simulink model "FsaeDynoFull"  (R2026a)
settings: Solver=FixedStepDiscrete  StopTime=t_stop  FixedStep=Ts  EnableMultiTasking=on
PreLoadFcn:
  | FsaeDynoFullData;
InitFcn:
  | FsaeDynoFullData;
values from neighbouring files (symbols this model uses):
  ce = 100    [FsaeDynoFullData.m]
  k_pre = 0.95    [FsaeDynoFullData.m]    (also in FsaeDynoFullPlot.m = evalin('base','k_pre'))
  Ki_id = Rs*wc_dut    (= 13.3454855924)    [FsaeDynoFullData.m]
  Ki_ids = Rs_y*wc_load    (= 47.1238898038)    [FsaeDynoFullData.m]
  Ki_iq = Rs*wc_dut    (= 13.3454855924)    [FsaeDynoFullData.m]
  Ki_iqs = Rs_y*wc_load    (= 47.1238898038)    [FsaeDynoFullData.m]
  Kp_id = Ld*wc_dut    (= 0.102541584213)    [FsaeDynoFullData.m]
  Kp_ids = Ld_y*wc_load    (= 0.204203522483)    [FsaeDynoFullData.m]
  Kp_iq = Lq*wc_dut    (= 0.105557513161)    [FsaeDynoFullData.m]
  Kp_iqs = Lq_y*wc_load    (= 0.204203522483)    [FsaeDynoFullData.m]
  Ld = 40.8e-6    (= 4.08e-05)    [FsaeDynoFullData.m]
  Lq = 42.0e-6    (= 4.2e-05)    [FsaeDynoFullData.m]
  p = 10    [FsaeDynoFullData.m]    (also in buildFsaeDynoFull.m = get_param(ss,'PortHandles'))
  psim = 0.03095    [FsaeDynoFullData.m]
  R_dis_dut = 1/G_dis_dut  - R_disRly    [FsaeDynoFullData.m]
  R_dis_load = 1/G_dis_load - R_disRly    [FsaeDynoFullData.m]
  R_pre_dut = fzero(@(R) preErr(R, Cdc_dut,  G_leak_dut  + G_disRlyOff), [1 1e5])    [FsaeDynoFullData.m]
  R_pre_load = fzero(@(R) preErr(R, Cdc_load, G_leak_load + G_disRlyOff), [1 1e5])    [FsaeDynoFullData.m]
  R_stby_dut = 50e3    (= 50000)    [FsaeDynoFullData.m]
  R_stby_load = 50e3    (= 50000)    [FsaeDynoFullData.m]
  t_InvEnDelay = 0.05    [FsaeDynoFullData.m]
  t_TSoff = t_test + 0.8 + 0.7    (= 2.7)    [FsaeDynoFullData.m]    (also in FsaeDynoFullPlot.m = evalin('base','t_TSoff'))
  Ts = 1e-5    (= 1e-05)    [FsaeDynoFullData.m]
  VbattMin = 50    [FsaeDynoFullData.m]
  VDC_VECT = Vnom*[0.9 1.0 1.1]    [FsaeDynoFullData.m]
  Vnom2 = 400    [FsaeDynoFullData.m]
libraries: nesl_utility x37, fl_lib x22, ee_lib x22, simulink x4, eeTransforms x2, batteryecm_lib x2, eePmsmFieldOrientedControl x1, eePmsmCurrentController x1, eePmsmCurrentReferenceGen x1, eePmsmTorqueEstimator x1, eePwmGeneratorTwoLevel x1
(part 2 of 2)

== system FsaeDynoFull/Sensing Torque IPMSM ==
  Elastic Coupling : fl_lib/Mechanical/Rotational Elements/Rotational Damper  D=ce N*m/(rad/s)  w_specify=off  w_priority=None  w=0 rad/s  w_nominal_specify=off  w_nominal_value=1  w_nominal_unit=rad/s  t_specify=off  t_priority=None  t=0 N*m  t_nominal_specify=off  t_nominal_value=1  t_nominal_unit=N*m
      settings: LogSimulationData=on
  Goto3 : Goto  TagVisibility=global
  Mechanical Rotational Reference1 : fl_lib/Mechanical/Rotational Elements/Mechanical Rotational Reference
  PS-Simulink Converter1 : nesl_utility/PS-Simulink Converter  PhysicalDomain=network_engine_domain  SubClassName=ps_output  LeftPortType=input  RightPortType=output  PseudoPeriodic=off  Frequencies=[]  VectorFormat=1-D array  Unit=rad/s  AffineConversion=off
  PS-Simulink Converter2 : nesl_utility/PS-Simulink Converter  PhysicalDomain=network_engine_domain  SubClassName=ps_output  LeftPortType=input  RightPortType=output  PseudoPeriodic=off  Frequencies=[]  VectorFormat=1-D array  Unit=rad  AffineConversion=off
  PS-Simulink Converter3 : nesl_utility/PS-Simulink Converter  PhysicalDomain=network_engine_domain  SubClassName=ps_output  LeftPortType=input  RightPortType=output  PseudoPeriodic=off  Frequencies=[]  VectorFormat=1-D array  Unit=N*m  AffineConversion=off
  Rotational Motion Sensor : fl_lib/Mechanical/Mechanical Sensors/Ideal Rotational Motion Sensor  reference=foundation.enum.MeasurementReference.difference  acceleration_port=false  velocity_port=true  position_port=true  wrap_angle=simscape.enum.onoff.off  offset=0 deg
  Torque Sensor : fl_lib/Mechanical/Mechanical Sensors/Ideal Torque Sensor
  R : PMIOPort  Side=Left
  C : PMIOPort  Port=2  Side=Right
  tag scope: Tq_meas=global, W=global
  wires:
  PS-Simulink Converter2/1 -> Goto3/1
  PS-Simulink Converter1/1 -> [W]
  PS-Simulink Converter3/1 -> [Tq_meas]
  connections:
  Mechanical Rotational Reference1/LConn1 -- Rotational Motion Sensor/RConn1
  Rotational Motion Sensor/RConn3 -- PS-Simulink Converter2/LConn1
  Rotational Motion Sensor/RConn2 -- PS-Simulink Converter1/LConn1
  Torque Sensor/RConn2 -- PS-Simulink Converter3/LConn1
  Torque Sensor/RConn1 -- Elastic Coupling/LConn1 -- Rotational Motion Sensor/LConn1
  Elastic Coupling/RConn1 -- C/RConn1
  Torque Sensor/LConn1 -- R/RConn1

== system FsaeDynoFull/Sensing Torque IPMSM1 ==
  PS-Simulink Converter3 : nesl_utility/PS-Simulink Converter  PhysicalDomain=network_engine_domain  SubClassName=ps_output  LeftPortType=input  RightPortType=output  PseudoPeriodic=off  Frequencies=[]  VectorFormat=1-D array  Unit=N*m  AffineConversion=off
  Torque Sensor : fl_lib/Mechanical/Mechanical Sensors/Ideal Torque Sensor
  C : PMIOPort  Side=Left
  R : PMIOPort  Port=2  Side=Right
  tag scope: Tq_asm=global
  wires:
  PS-Simulink Converter3/1 -> [Tq_asm]
  connections:
  C/RConn1 -- Torque Sensor/RConn1
  R/RConn1 -- Torque Sensor/LConn1
  Torque Sensor/RConn2 -- PS-Simulink Converter3/LConn1

== system FsaeDynoFull/Sensing current1 ==
  Current Sensor : ee_lib/Sensors & Transducers/Current Sensor (Three-Phase)  port_option=ee.enum.threePhasePort.composite
  PS-Simulink Converter : nesl_utility/PS-Simulink Converter  PhysicalDomain=network_engine_domain  SubClassName=ps_output  LeftPortType=input  RightPortType=output  PseudoPeriodic=off  Frequencies=[]  VectorFormat=1-D array  Unit=A  AffineConversion=off
  1 : PMIOPort  Side=Left
  2 : PMIOPort  Port=2  Side=Right
  tag scope: I_ABC=global
  wires:
  PS-Simulink Converter/1 -> [I_ABC]
  connections:
  1/RConn1 -- Current Sensor/LConn1
  2/RConn1 -- Current Sensor/RConn2
  Current Sensor/RConn1 -- PS-Simulink Converter/LConn1

== system FsaeDynoFull/Sensing current2 ==
  Current Sensor : ee_lib/Sensors & Transducers/Current Sensor (Three-Phase)  port_option=ee.enum.threePhasePort.composite
  PS-Simulink Converter : nesl_utility/PS-Simulink Converter  PhysicalDomain=network_engine_domain  SubClassName=ps_output  LeftPortType=input  RightPortType=output  PseudoPeriodic=off  Frequencies=[]  VectorFormat=1-D array  Unit=A  AffineConversion=off
  1 : PMIOPort  Side=Left
  2 : PMIOPort  Port=2  Side=Right
  tag scope: I_ABC2=global
  wires:
  PS-Simulink Converter/1 -> [I_ABC2]
  connections:
  Current Sensor/RConn1 -- PS-Simulink Converter/LConn1
  2/RConn1 -- Current Sensor/RConn2
  1/RConn1 -- Current Sensor/LConn1

== system FsaeDynoFull/Sensing voltage1 ==
  PS-Simulink Converter4 : nesl_utility/PS-Simulink Converter  PhysicalDomain=network_engine_domain  SubClassName=ps_output  LeftPortType=input  RightPortType=output  PseudoPeriodic=off  Frequencies=[]  VectorFormat=1-D array  Unit=V  AffineConversion=off
  Voltage Sensor : fl_lib/Electrical/Electrical Sensors/Voltage Sensor
  + : PMIOPort  Side=Left
  - : PMIOPort  Port=2  Side=Right
  tag scope: Vdc=global
  wires:
  PS-Simulink Converter4/1 -> [Vdc]
  connections:
  Voltage Sensor/LConn1 -- +/RConn1
  Voltage Sensor/RConn2 -- -/RConn1
  PS-Simulink Converter4/LConn1 -- Voltage Sensor/RConn1

== system FsaeDynoFull/Sensing voltage2 ==
  PS-Simulink Converter4 : nesl_utility/PS-Simulink Converter  PhysicalDomain=network_engine_domain  SubClassName=ps_output  LeftPortType=input  RightPortType=output  PseudoPeriodic=off  Frequencies=[]  VectorFormat=1-D array  Unit=V  AffineConversion=off
  Voltage Sensor : fl_lib/Electrical/Electrical Sensors/Voltage Sensor
  + : PMIOPort  Side=Left
  - : PMIOPort  Port=2  Side=Right
  tag scope: Vdc2=global
  wires:
  PS-Simulink Converter4/1 -> [Vdc2]
  connections:
  PS-Simulink Converter4/LConn1 -- Voltage Sensor/RConn1
  Voltage Sensor/RConn2 -- -/RConn1
  Voltage Sensor/LConn1 -- +/RConn1

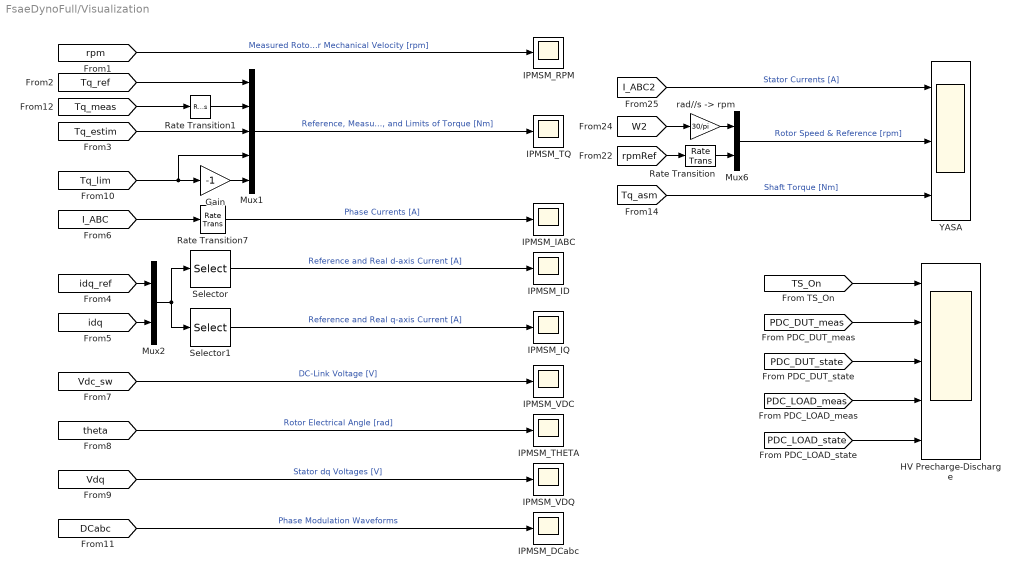
== system FsaeDynoFull/Visualization ==
  Gain : Gain  Gain=-1
  HV Precharge-Discharge : Scope  NumInputPorts=5
      settings: TimeSpan=t_stop  ActiveDisplayYMinimum=-0.12499999999999997  ActiveDisplayYMaximum=1.125
  IPMSM_DCabc : Scope
      settings: ActiveDisplayYMinimum=-1.20582  ActiveDisplayYMaximum=1.20582
  IPMSM_IABC : Scope
      settings: ActiveDisplayYMinimum=-467.55489  ActiveDisplayYMaximum=466.19547  DataLoggingVariableName=ScopeData5
  IPMSM_ID : Scope
      settings: ActiveDisplayYMinimum=-119.30465229514377  ActiveDisplayYMaximum=159.91436095303817  DataLoggingSaveFormat=Array
  IPMSM_IQ : Scope
      settings: ActiveDisplayYMinimum=-543.15194036102753  ActiveDisplayYMaximum=577.1433935962757  DataLoggingVariableName=ScopeData2  DataLoggingSaveFormat=Array
  IPMSM_RPM : Scope
      settings: ActiveDisplayYMinimum=-293.41664  ActiveDisplayYMaximum=2640.63347
  IPMSM_THETA : Scope
      settings: ActiveDisplayYMinimum=-0.7854  ActiveDisplayYMaximum=7.06858  DataLoggingVariableName=ScopeData7
  IPMSM_TQ : Scope
      settings: ActiveDisplayYMinimum=-258.76977  ActiveDisplayYMaximum=278.92486  DataLoggingVariableName=ScopeData2
  IPMSM_VDC : Scope
      settings: ActiveDisplayYMinimum=-37.00643  ActiveDisplayYMaximum=365.23613  DataLoggingVariableName=ScopeData6
  IPMSM_VDQ : Scope
      settings: ActiveDisplayYMinimum=-165.01838  ActiveDisplayYMaximum=203.34651  DataLoggingVariableName=ScopeData8
  Mux1 : Mux  Inputs=5
  Mux2 : Mux  Inputs=2
  Mux6 : Mux  Inputs=2
  Rate Transition : RateTransition
  Rate Transition1 : RateTransition
  Rate Transition7 : RateTransition  OutPortSampleTime=1e-4
  Selector : Selector  InputPortWidth=4  IndexOptions=Index vector (dialog)  Indices=[1 3]  OutputSizes=1
  Selector1 : Selector  InputPortWidth=4  IndexOptions=Index vector (dialog)  Indices=[2 4]  OutputSizes=1
  YASA : Scope  NumInputPorts=3
      settings: ActiveDisplayYMinimum=-633.40768  ActiveDisplayYMaximum=631.34381  DataLoggingVariableName=ScopeData2
  "rad//s -> rpm" : Gain  Gain=30/pi
  wires:
  [rpm] -> IPMSM_RPM/1  "Measured Rotor Mechanical Velocity [rpm]"
  Mux1/1 -> IPMSM_TQ/1  "Reference, Measured, Estim, and Limits of Torque [Nm]"
  [Tq_ref] -> Mux1/1
  [I_ABC] -> Rate Transition7/1
  [Vdc_sw] -> IPMSM_VDC/1  "DC-Link Voltage [V]"
  [theta] -> IPMSM_THETA/1  "Rotor Electrical Angle [rad]"
  [Vdq] -> IPMSM_VDQ/1  "Stator dq Voltages [V]"
  [Tq_lim] -> Mux1/4, Gain/1
  [DCabc] -> IPMSM_DCabc/1  "Phase Modulation Waveforms"
  [W2] -> "rad//s -> rpm"/1
  [I_ABC2] -> YASA/1  "Stator Currents [A]"
  Mux6/1 -> YASA/2  "Rotor Speed & Reference [rpm]"
  [rpmRef] -> Rate Transition/1
  "rad//s -> rpm"/1 -> Mux6/1
  Rate Transition/1 -> Mux6/2
  Rate Transition7/1 -> IPMSM_IABC/1  "Phase Currents [A]"
  Selector1/1 -> IPMSM_IQ/1  "Reference and Real q-axis Current [A]"
  [idq_ref] -> Mux2/1
  Selector/1 -> IPMSM_ID/1  "Reference and Real d-axis Current [A]"
  Mux2/1 -> Selector1/1, Selector/1
  [idq] -> Mux2/2
  [Tq_meas] -> Rate Transition1/1
  Gain/1 -> Mux1/5
  Rate Transition1/1 -> Mux1/2
  [Tq_estim] -> Mux1/3
  [Tq_asm] -> YASA/3  "Shaft Torque [Nm]"
  [TS_On] -> HV Precharge-Discharge/1
  [PDC_DUT_meas] -> HV Precharge-Discharge/2
  [PDC_DUT_state] -> HV Precharge-Discharge/3
  [PDC_LOAD_meas] -> HV Precharge-Discharge/4
  [PDC_LOAD_state] -> HV Precharge-Discharge/5

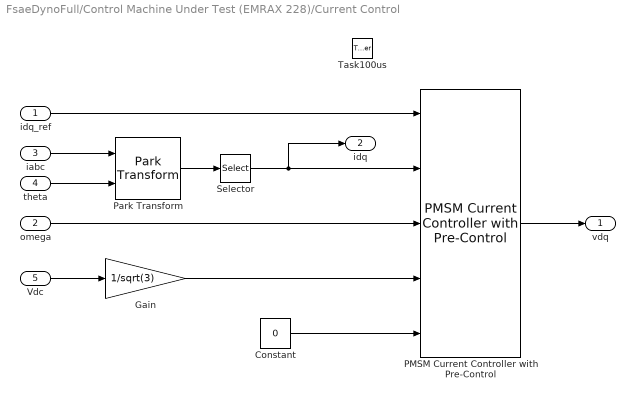
== system FsaeDynoFull/Control Machine Under Test (EMRAX 228)/Current Control ==
  idq_ref : Inport
  omega : Inport  Port=2
  iabc : Inport  Port=3
  theta : Inport  Port=4
  Vdc : Inport  Port=5
  Task100us : TriggerPort  TriggerType=function-call  VariantControl=Variant  PortDimensions=1
  Constant : Constant  Value=0  SampleTime=-1
  Gain : Gain  Gain=1/sqrt(3)
  PMSM Current Controller with Pre-Control : eePmsmCurrentController/PMSM Current Controller with Pre-Control  Kp_id=Kp_id  Ki_id=Ki_id  Kaw_id=Ki_id/Kp_id  Kp_iq=Kp_iq  Ki_iq=Ki_iq  Kaw_iq=Ki_iq/Kp_iq  Ts=-1  Tsd=Tsi  AxisPrio=Q-axis  ActZC=on  ActFF=on  idVect=[-200, 0, 200]  iqVect=[-200, 0, 200]  LdMatrix=Ld * ones(3, 3)  LqMatrix=Lq * ones(3, 3)  psimMatrix=psim * ones(3, 3)
  Park Transform : eeTransforms/Park Transform  AxisAlignment=Q-axis  PowerInvariant=off
  Selector : Selector  InputPortWidth=3  IndexOptions=Index vector (dialog)  Indices=[1 2]  OutputSizes=1
  vdq : Outport  VectorParamsAs1DForOutWhenUnconnected=off
  idq : Outport  Port=2  VectorParamsAs1DForOutWhenUnconnected=off
  wires:
  idq_ref/1 -> PMSM Current Controller with Pre-Control/1
  iabc/1 -> Park Transform/1
  theta/1 -> Park Transform/2
  omega/1 -> PMSM Current Controller with Pre-Control/3
  Vdc/1 -> Gain/1
  Gain/1 -> PMSM Current Controller with Pre-Control/4
  Constant/1 -> PMSM Current Controller with Pre-Control/5
  PMSM Current Controller with Pre-Control/1 -> vdq/1
  Selector/1 -> idq/1, PMSM Current Controller with Pre-Control/2
  Park Transform/1 -> Selector/1

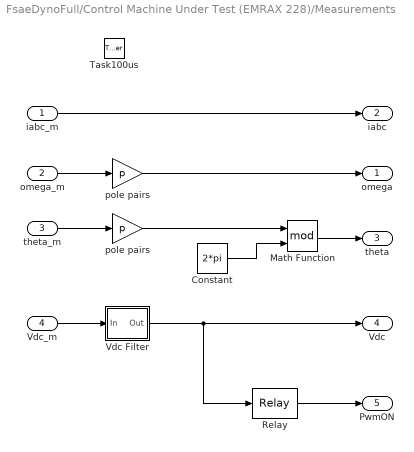
== system FsaeDynoFull/Control Machine Under Test (EMRAX 228)/Measurements ==
  iabc_m : Inport
  omega_m : Inport  Port=2
  theta_m : Inport  Port=3
  Vdc_m : Inport  Port=4
  Task100us : TriggerPort  TriggerType=function-call  VariantControl=Variant  PortDimensions=1
  Constant : Constant  Value=2*pi  SampleTime=-1
  Math Function : Math  Operator=mod  SignedPower=on
  Relay : Relay  OnSwitchValue=VDC_VECT(1)  OffSwitchValue=0.5*VDC_VECT(1)
  Vdc Filter : Subsystem  mask(Discrete first-order filter (Low-pass)){T=0.005, Ts=1e-4}
      mask prompts: T "Time constant (s):"; Ts "Sample time (s):"
      mask help: This block implements a discrete low-pass filter. To calculate the coefficients, the block discretises a continuous low-pass filter using the Tustin method.
      mask init:
      | num = [ Ts/(2*T + Ts), Ts/(2*T + Ts)];
      | den = [ 1, -(2*T - Ts)/(2*T + Ts)];
  pole pairs : Gain  Gain=p
  "pole pairs " : Gain  Gain=p
  omega : Outport  VectorParamsAs1DForOutWhenUnconnected=off
  iabc : Outport  Port=2  VectorParamsAs1DForOutWhenUnconnected=off
  theta : Outport  Port=3  VectorParamsAs1DForOutWhenUnconnected=off
  Vdc : Outport  Port=4  VectorParamsAs1DForOutWhenUnconnected=off
  PwmON : Outport  Port=5  VectorParamsAs1DForOutWhenUnconnected=off
  wires:
  pole pairs/1 -> omega/1
  theta_m/1 -> "pole pairs "/1
  omega_m/1 -> pole pairs/1
  iabc_m/1 -> iabc/1
  "pole pairs "/1 -> Math Function/1
  Constant/1 -> Math Function/2
  Math Function/1 -> theta/1
  Vdc_m/1 -> Vdc Filter/1(In)
  Relay/1 -> PwmON/1
  Vdc Filter/1(Out) -> Relay/1, Vdc/1

== system FsaeDynoFull/Control Machine Under Test (EMRAX 228)/Outer Loop Control ==
  TqRequest : Inport
  idq : Inport  Port=2
  we : Inport  Port=3
  Vdc : Inport  Port=4
  Task1ms : TriggerPort  TriggerType=function-call  VariantControl=Variant  PortDimensions=1
  PMSM Current Reference Generator : eePmsmCurrentReferenceGen/PMSM Current Reference Generator  Vnom=Vnom  Pmax=Pmax  Tmax=Tmax  Ts=-1  RefType=Automatically generated lookup-table  rpmVec=RPM_VECT  TqVec=TQ_VECT  VdcVec=VDC_VECT  PWMMode=SVM: space vector modulation  ModFactor=1  idMatrix=ID_MAP  iqMatrix=IQ_MAP  p=p  psim=psim  Ld=Ld  Lq=Lq  Rs=Rs  RefExpEnable=0
  PMSM Torque Estimator : eePmsmTorqueEstimator/PMSM Torque Estimator  ParamType=Constant parameters  p=p  idVect=[-200, 200]  iqVect=[-200, 200]  LdMatrix=0.0002 * ones(2, 2)  LqMatrix=0.0002 * ones(2, 2)  psimMatrix=0.04 * ones(2, 2)  Ld=Ld  Lq=Lq  psim=psim  Ts=-1
  elec->mech : Gain  Gain=1/p
  idq_ref : Outport  VectorParamsAs1DForOutWhenUnconnected=off
  Tq_ref : Outport  Port=2  VectorParamsAs1DForOutWhenUnconnected=off
  Tq_lim : Outport  Port=3  VectorParamsAs1DForOutWhenUnconnected=off
  Tq_estim : Outport  Port=4  VectorParamsAs1DForOutWhenUnconnected=off
  wires:
  PMSM Current Reference Generator/1 -> idq_ref/1
  PMSM Torque Estimator/1 -> Tq_estim/1
  idq/1 -> PMSM Torque Estimator/1
  elec->mech/1 -> PMSM Current Reference Generator/2
  Vdc/1 -> PMSM Current Reference Generator/3
  PMSM Current Reference Generator/2 -> Tq_ref/1
  TqRequest/1 -> PMSM Current Reference Generator/1
  we/1 -> elec->mech/1
  PMSM Current Reference Generator/3 -> Tq_lim/1

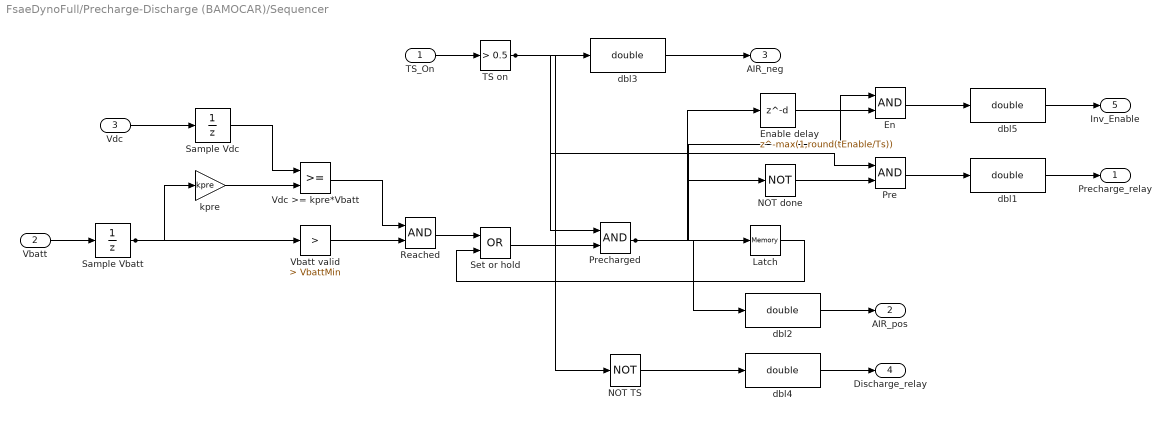
== system FsaeDynoFull/Precharge-Discharge (BAMOCAR)/Sequencer ==
  TS_On : Inport
  Vbatt : Inport  Port=2
  Vdc : Inport  Port=3
  En : Logic  AllPortsSameDT=off  OutDataTypeStr=boolean
  Enable delay : Delay  DelayLength=max(1,round(tEnable/Ts))  InitialCondition=0  SampleTime=Ts
  Latch : Memory
  NOT TS : Logic  Operator=NOT  AllPortsSameDT=off  OutDataTypeStr=boolean
  NOT done : Logic  Operator=NOT  AllPortsSameDT=off  OutDataTypeStr=boolean
  Pre : Logic  AllPortsSameDT=off  OutDataTypeStr=boolean
  Precharged : Logic  AllPortsSameDT=off  OutDataTypeStr=boolean
  Reached : Logic  AllPortsSameDT=off  OutDataTypeStr=boolean
  Sample Vbatt : UnitDelay  SampleTime=Ts
  Sample Vdc : UnitDelay  SampleTime=Ts
  Set or hold : Logic  Operator=OR  AllPortsSameDT=off  OutDataTypeStr=boolean
  TS on : simulink/Logic and Bit Operations/Compare To Constant  relop=>  const=0.5  OutDataTypeStr=boolean
  Vbatt valid : simulink/Logic and Bit Operations/Compare To Constant  relop=>  const=VbattMin  OutDataTypeStr=boolean
  Vdc >= kpre*Vbatt : RelationalOperator  OutDataTypeStr=boolean  RndMeth=Simplest  InputSameDT=off
  dbl{1..5} (5 alike) : DataTypeConversion  OutDataTypeStr=double  SaturateOnIntegerOverflow=off  RndMeth=Floor
  kpre : Gain  Gain=kpre
  Precharge_relay : Outport
  AIR_pos : Outport  Port=2
  AIR_neg : Outport  Port=3
  Discharge_relay : Outport  Port=4
  Inv_Enable : Outport  Port=5
  wires:
  Vbatt/1 -> Sample Vbatt/1
  Sample Vbatt/1 -> Vbatt valid/1, kpre/1
  Vdc/1 -> Sample Vdc/1
  Sample Vdc/1 -> Vdc >= kpre*Vbatt/1
  Vdc >= kpre*Vbatt/1 -> Reached/1
  kpre/1 -> Vdc >= kpre*Vbatt/2
  Vbatt valid/1 -> Reached/2
  TS_On/1 -> TS on/1
  Reached/1 -> Set or hold/1
  Pre/1 -> dbl1/1
  TS on/1 -> Pre/1, NOT TS/1, dbl3/1, Precharged/1
  Set or hold/1 -> Precharged/2
  dbl3/1 -> AIR_neg/1
  Precharged/1 -> En/1, Latch/1, Enable delay/1, dbl2/1, NOT done/1
  NOT TS/1 -> dbl4/1
  Enable delay/1 -> En/2
  NOT done/1 -> Pre/2
  Latch/1 -> Set or hold/2
  dbl2/1 -> AIR_pos/1
  dbl4/1 -> Discharge_relay/1
  En/1 -> dbl5/1
  dbl5/1 -> Inv_Enable/1
  dbl1/1 -> Precharge_relay/1

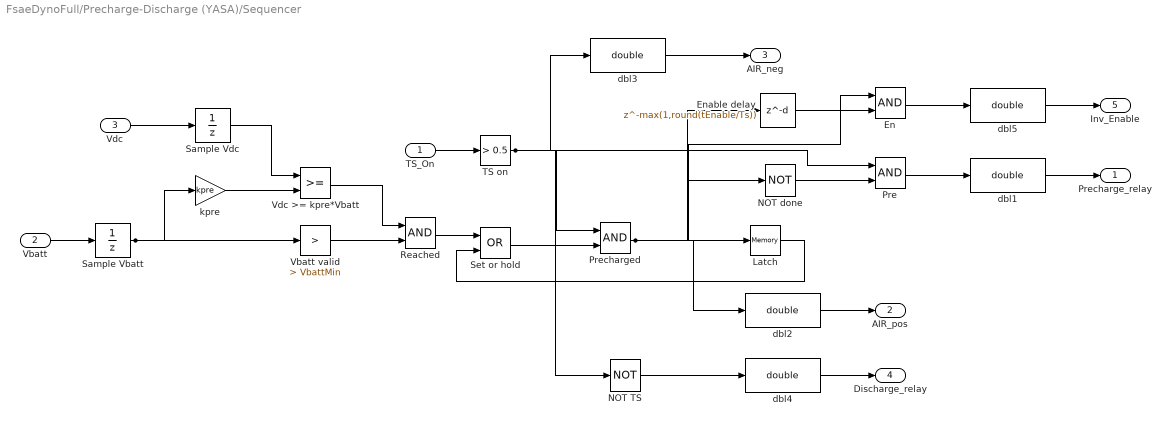
== system FsaeDynoFull/Precharge-Discharge (YASA)/Sequencer ==
  TS_On : Inport
  Vbatt : Inport  Port=2
  Vdc : Inport  Port=3
  En : Logic  AllPortsSameDT=off  OutDataTypeStr=boolean
  Enable delay : Delay  DelayLength=max(1,round(tEnable/Ts))  InitialCondition=0  SampleTime=Ts
  Latch : Memory
  NOT TS : Logic  Operator=NOT  AllPortsSameDT=off  OutDataTypeStr=boolean
  NOT done : Logic  Operator=NOT  AllPortsSameDT=off  OutDataTypeStr=boolean
  Pre : Logic  AllPortsSameDT=off  OutDataTypeStr=boolean
  Precharged : Logic  AllPortsSameDT=off  OutDataTypeStr=boolean
  Reached : Logic  AllPortsSameDT=off  OutDataTypeStr=boolean
  Sample Vbatt : UnitDelay  SampleTime=Ts
  Sample Vdc : UnitDelay  SampleTime=Ts
  Set or hold : Logic  Operator=OR  AllPortsSameDT=off  OutDataTypeStr=boolean
  TS on : simulink/Logic and Bit Operations/Compare To Constant  relop=>  const=0.5  OutDataTypeStr=boolean
  Vbatt valid : simulink/Logic and Bit Operations/Compare To Constant  relop=>  const=VbattMin  OutDataTypeStr=boolean
  Vdc >= kpre*Vbatt : RelationalOperator  OutDataTypeStr=boolean  RndMeth=Simplest  InputSameDT=off
  dbl{1..5} (5 alike) : DataTypeConversion  OutDataTypeStr=double  SaturateOnIntegerOverflow=off  RndMeth=Floor
  kpre : Gain  Gain=kpre
  Precharge_relay : Outport
  AIR_pos : Outport  Port=2
  AIR_neg : Outport  Port=3
  Discharge_relay : Outport  Port=4
  Inv_Enable : Outport  Port=5
  wires:
  Latch/1 -> Set or hold/2
  Vbatt/1 -> Sample Vbatt/1
  Pre/1 -> dbl1/1
  Sample Vbatt/1 -> Vbatt valid/1, kpre/1
  Vbatt valid/1 -> Reached/2
  Vdc/1 -> Sample Vdc/1
  Sample Vdc/1 -> Vdc >= kpre*Vbatt/1
  Precharged/1 -> En/1, NOT done/1, Latch/1, Enable delay/1, dbl2/1
  TS_On/1 -> TS on/1
  Vdc >= kpre*Vbatt/1 -> Reached/1
  kpre/1 -> Vdc >= kpre*Vbatt/2
  Reached/1 -> Set or hold/1
  TS on/1 -> Pre/1, Precharged/1, NOT TS/1, dbl3/1
  Set or hold/1 -> Precharged/2
  dbl3/1 -> AIR_neg/1
  NOT TS/1 -> dbl4/1
  Enable delay/1 -> En/2
  NOT done/1 -> Pre/2
  dbl2/1 -> AIR_pos/1
  dbl4/1 -> Discharge_relay/1
  En/1 -> dbl5/1
  dbl5/1 -> Inv_Enable/1
  dbl1/1 -> Precharge_relay/1

== system FsaeDynoFull/Control Machine Under Test (EMRAX 228)/Measurements/Vdc Filter ==
  In : Inport
  Discrete Transfer Fcn : DiscreteTransferFcn  Numerator=num  Denominator=den
  Out : Outport  VectorParamsAs1DForOutWhenUnconnected=off
  wires:
  Discrete Transfer Fcn/1 -> Out/1
  In/1 -> Discrete Transfer Fcn/1

== stateflow chart FsaeDynoFull/Control Machine Under Test (EMRAX 228)/Task Scheduler ==
  (default) -> (junction 23) : CLK_50us
  (junction 23) -> (junction 17)
  (junction 17) -> (junction 22) [order 2]
  (junction 17) -> (junction 22) [order 1] : [cnt%%2==0]{Task_100us_1;}
  (junction 22) -> (junction 18) [order 2]
  (junction 22) -> (junction 18) [order 1] : [cnt%%2==0]{Task_100us_2;}
  (junction 18) -> (junction 21) [order 2]
  (junction 18) -> (junction 21) [order 1] : [cnt%%20==0]{Task_1ms_1;}
  (junction 21) -> (junction 34) [order 2]
  (junction 21) -> (junction 16) [order 1] : [1]{cnt++;}
  data: cnt local int32
  events: Task_100us_1 output FUNCTION_CALL_EVENT; Task_100us_2 output FUNCTION_CALL_EVENT; Task_1ms_1 output FUNCTION_CALL_EVENT; CLK_50us input FUNCTION_CALL_EVENT
